simulink model "Tracking"  (R2024b)
settings: Solver=VariableStepAuto  StartTime=0.0  StopTime=1000  RelTol=1e-3
values from neighbouring files (symbols this model uses):
  A = A + DCM_out_slew(:,:,jj)    [sadcode.m]
  a = 6899750    [sadcode.m]
  Area_vect = [3;3;3;3;1;1;1;1;1;1]    [sadcode.m]
  C_d = 2.2    [sadcode.m]
  e = 0.0005895    [sadcode.m]
  G = 6.67e-11    [sadcode.m]
  g = [g1_0 g2_0 g3_0 g4_0 g5_0 g6_0 g7_0 g8_0 g9_0 g10_0  g11_0  g12_0  g13_0 ... (first row only)    [IGRF13.m]
  h = [h1_0 h2_0 h3_0 h4_0 h5_0 h6_0 h7_0 h8_0 h9_0 h10_0  h11_0  h12_0  h13_0 ... (first row only)    [IGRF13.m]
  I = diag([Ix,Iy,Iz])    [sadcode.m]
  i = deg2rad(5.0097)    [sadcode.m]
  Ix = 4.208e11*10^(-3-6)    (= 420.8)    [sadcode.m]
  Iy = 4.922e12*10^(-3-6)    (= 4922)    [sadcode.m]
  Iz = 4.399e12*10^(-3-6)    (= 4399)    [sadcode.m]
  J_b = [1 ; 18 ; 5]    [sadcode.m]
  K_slew = diag(K_slew)    [sadcode.m]
  M = 5.97219e24    (= 5.97219e+24)    [sadcode.m]
  Mount = [0 0 1 0 1 0]    [sadcode.m]
  mu = G*M    (= 398345073000000)    [sadcode.m]
  n = sqrt(mu/a^3)    [sadcode.m]
  N_b = [0,0,+1; 0,0,-1; 0,0,1; 0,0,-1;1,0,0 ; -1,0,0; 0,1,0; 0,-1,0; 0,0,1; 0,0,-1]    [sadcode.m]
  n_face = length(rho_s)    [sadcode.m]
  p = a * (1 - e^2)    (= 6899747.60227)    [sadcode.m]
  q = abs(q(:,1))    [sadcode.m]
  R_f = [2.5,0,0; 2.5,0,0; -2.5,0,0; -2.5,0,0; 1,0,0; -1,0,0; 0,1,0; 0,-1,0; 0,0,1; 0,0,-1]    [sadcode.m]
  R_sun = 149597870700    [sadcode.m]
  rho = 3.13e-13    [sadcode.m]
  theta0 = theta0_slew(jj)    [sadcode.m]
  w0x = w_out_slew(1,jj)    [sadcode.m]
  w0y = w_out_slew(2,jj)    [sadcode.m]
  w0z = w_out_slew(3,jj)    [sadcode.m]
  w_earth = 2*pi/(24*3600)    (= 7.27220521664e-05)    [sadcode.m]
undefined symbols (not defined in the file or in its folder): DiscIntNeverNeededParam
libraries: simulink x4
(part 2 of 2)

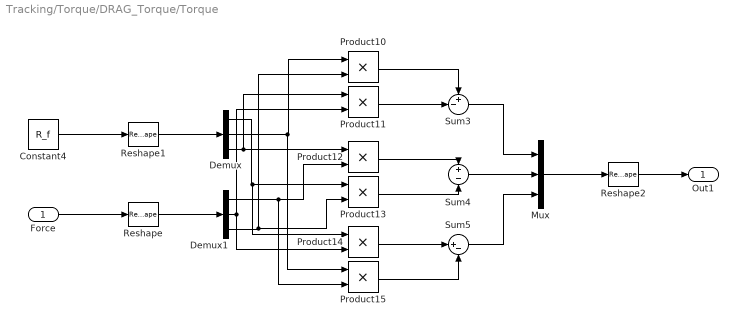
== system Tracking/Torque/DRAG_Torque/Torque ==
  Force : Inport
  Constant4 : Constant  Value=R_f
  Demux : Demux  Outputs=3
  Demux1 : Demux  Outputs=3
  Mux : Mux  Inputs=3
  Product{10..15} (6 alike) : Product
  Reshape : Reshape  OutputDimensionality=Column vector (2-D)
  Reshape1 : Reshape  OutputDimensionality=Column vector (2-D)
  Reshape2 : Reshape  OutputDimensionality=Customize  OutputDimensions=[n_face,3]
  Sum3 : Sum  Inputs=+-|
  Sum4 : Sum  Inputs=+|-
  Sum5 : Sum  Inputs=|+-
  Out1 : Outport
  wires:
  Product12/1 -> Sum4/1
  Demux1/1 -> Product15/2, Product12/2
  Reshape2/1 -> Out1/1
  Demux/1 -> Product14/1, Product13/1
  Sum5/1 -> Mux/3
  Constant4/1 -> Reshape1/1
  Mux/1 -> Reshape2/1
  Reshape/1 -> Demux1/1
  Demux/3 -> Product12/1, Product11/1
  Demux1/3 -> Product13/2, Product10/2
  Force/1 -> Reshape/1
  Product13/1 -> Sum4/2
  Reshape1/1 -> Demux/1
  Sum3/1 -> Mux/1
  Product11/1 -> Sum3/2
  Demux1/2 -> Product11/2, Product14/2
  Demux/2 -> Product15/1, Product10/1
  Sum4/1 -> Mux/2
  Product14/1 -> Sum5/1
  Product10/1 -> Sum3/1
  Product15/1 -> Sum5/2

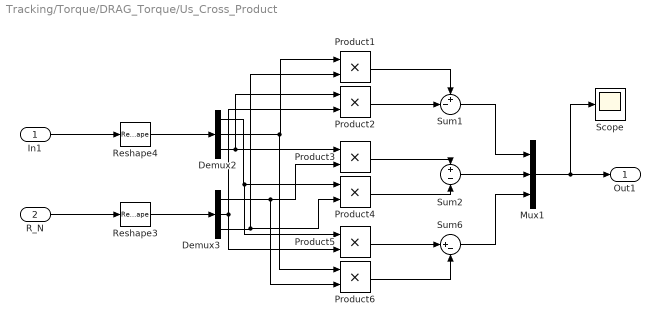
== system Tracking/Torque/DRAG_Torque/Us_Cross_Product  ==
  In1 : Inport
  R_N : Inport  Port=2
  Demux2 : Demux  Outputs=3
  Demux3 : Demux  Outputs=3
  Mux1 : Mux  Inputs=3
  Product{1..6} (6 alike) : Product
  Reshape3 : Reshape  OutputDimensionality=Column vector (2-D)
  Reshape4 : Reshape  OutputDimensionality=Column vector (2-D)
  Scope : Scope
  Sum1 : Sum  Inputs=+-|
  Sum2 : Sum  Inputs=+|-
  Sum6 : Sum  Inputs=|+-
  Out1 : Outport
  wires:
  Reshape3/1 -> Demux3/1
  Reshape4/1 -> Demux2/1
  Demux3/1 -> Product6/2, Product3/2
  Demux2/1 -> Product5/1, Product4/1
  Demux3/3 -> Product4/2, Product1/2
  Sum2/1 -> Mux1/2
  Product6/1 -> Sum6/2
  Sum6/1 -> Mux1/3
  Demux2/2 -> Product6/1, Product1/1
  Demux3/2 -> Product2/2, Product5/2
  Product3/1 -> Sum2/1
  Product2/1 -> Sum1/2
  Product4/1 -> Sum2/2
  Demux2/3 -> Product3/1, Product2/1
  Mux1/1 -> Scope/1, Out1/1
  Product1/1 -> Sum1/1
  Sum1/1 -> Mux1/1
  Product5/1 -> Sum6/1
  In1/1 -> Reshape4/1
  R_N/1 -> Reshape3/1

== system Tracking/Torque/DRAG_Torque/V_vect ==
  Theta : Inport
  Constant : Constant  Value=sqrt(mu/p)
  Constant1 : Constant  Value=e
  Constant2 : Constant  Value=0
  Constant3 : Constant  Value=Rot'
  Gain : Gain  Gain=-1
  Mux : Mux  Inputs=3
  Product : Product
  Product1 : Product  Multiplication=Matrix(*)
  Sin : Trigonometry
  Sin1 : Trigonometry  Operator=cos
  Sum : Sum  Inputs=|++
  Out1 : Outport
  wires:
  Constant/1 -> Product/1
  Mux/1 -> Product/2
  Sin/1 -> Gain/1
  Gain/1 -> Mux/1
  Sin1/1 -> Sum/1
  Sum/1 -> Mux/2
  Constant1/1 -> Sum/2
  Theta/1 -> Sin1/1, Sin/1
  Constant2/1 -> Mux/3
  Constant3/1 -> Product1/1
  Product1/1 -> Out1/1
  Product/1 -> Product1/2

== system Tracking/Torque/GG_Torque/A_BL1 ==
  A_LN : Inport
  A_BN : Inport  Port=2
  Matrix Multiply : Product  Multiplication=Matrix(*)
  Transpose : Math  Operator=transpose
  A_BL : Outport
  wires:
  Transpose/1 -> Matrix Multiply/2
  A_LN/1 -> Transpose/1
  Matrix Multiply/1 -> A_BL/1  "A_BL"
  A_BN/1 -> Matrix Multiply/1

== system Tracking/Torque/GG_Torque/GG_Torque_calc ==
  In1 : Inport
  |R| : Inport  Port=2
  Constant : Constant  Value=G*M
  Constant1 : Constant  Value=3
  Demux : Demux  Outputs=3
  Gain : Gain  Gain=-3
  Multiply3 : Gain  Gain=(Iy-Iz)
  Multiply4 : Gain  Gain=(-Ix+Iz)
  Multiply5 : Gain  Gain=(-Iy+Ix)
  Mux : Mux  Inputs=3
  Product3 : Product  Inputs=***
  Product4 : Product  Inputs=***
  Product5 : Product  Inputs=***
  Product6 : Product  Inputs=*/
  Scope : Scope
  Square : Math  Operator=pow
  GG_Torque : Outport
  wires:
  Multiply3/1 -> Mux/1
  Mux/1 -> GG_Torque/1
  Multiply4/1 -> Mux/2
  In1/1 -> Demux/1
  Product3/1 -> Multiply3/1
  Gain/1 -> Product5/1, Product4/1, Product3/1
  Demux/2 -> Product3/2, Product5/2
  Demux/3 -> Product3/3, Product4/3
  Product4/1 -> Multiply4/1
  Demux/1 -> Product4/2, Product5/3
  Product5/1 -> Multiply5/1
  Product6/1 -> Gain/1
  Constant/1 -> Product6/1
  |R|/1 -> Square/1
  Constant1/1 -> Square/2
  Square/1 -> Scope/1, Product6/2
  Multiply5/1 -> Mux/3

== system Tracking/Torque/GG_Torque/Subsystem ==
  A_BL : Inport
  Constant1 : Constant  Value=[1;0;0]
  Matrix Multiply3 : Product  Multiplication=Matrix(*)
  c_vector : Outport
  wires:
  Constant1/1 -> Matrix Multiply3/2
  Matrix Multiply3/1 -> c_vector/1  "c_vector"
  A_BL/1 -> Matrix Multiply3/1

== system Tracking/Torque/MAG_Torque/Us_Cross_Product ==
  In1 : Inport
  In2 : Inport  Port=2
  Demux2 : Demux  Outputs=3
  Demux3 : Demux  Outputs=3
  Mux1 : Mux  Inputs=3
  Product{1..6} (6 alike) : Product
  Reshape3 : Reshape  OutputDimensionality=Column vector (2-D)
  Reshape4 : Reshape  OutputDimensionality=Column vector (2-D)
  Sum1 : Sum  Inputs=+-|
  Sum2 : Sum  Inputs=+|-
  Sum6 : Sum  Inputs=|+-
  Out1 : Outport
  wires:
  Reshape3/1 -> Demux3/1
  Reshape4/1 -> Demux2/1
  Demux3/1 -> Product6/2, Product3/2
  Demux2/1 -> Product5/1, Product4/1
  Demux3/3 -> Product4/2, Product1/2
  Sum2/1 -> Mux1/2
  Product6/1 -> Sum6/2
  Sum6/1 -> Mux1/3
  Demux2/2 -> Product6/1, Product1/1
  Demux3/2 -> Product2/2, Product5/2
  Product3/1 -> Sum2/1
  Product2/1 -> Sum1/2
  Product4/1 -> Sum2/2
  Demux2/3 -> Product3/1, Product2/1
  Mux1/1 -> Out1/1
  Product1/1 -> Sum1/1
  Sum1/1 -> Mux1/1
  Product5/1 -> Sum6/1
  In1/1 -> Reshape4/1
  In2/1 -> Reshape3/1

== system Tracking/Torque/DRAG_Torque/Force/normalize2 ==
  vector : Inport
  Demux : Demux  Outputs=3
  Product : Product  Inputs=*/
  Square : Math  Operator=square
  Square Root : Sqrt
  Square1 : Math  Operator=square
  Square2 : Math  Operator=square
  Sum : Sum  Inputs=+++
  vers : Outport
  norm : Outport  Port=2
  wires:
  Square Root/1 -> norm/1, Product/2
  Demux/3 -> Square2/1
  Square2/1 -> Sum/3
  Square/1 -> Sum/1
  Square1/1 -> Sum/2
  Demux/1 -> Square/1
  Sum/1 -> Square Root/1
  vector/1 -> Product/1, Demux/1
  Demux/2 -> Square1/1
  Product/1 -> vers/1

== matlab function Tracking/Subsystem5/pseudoinverse ==
  data: u input; y output
function y = fcn(u)
A = u;
% Soluzione con norma minima
x = pinv(A) ;
y = x;

== matlab function Tracking/Torque/MAG_Torque/MATLAB Function1 ==
  data: r_N input; B_N output; t input; g input; h input
function B_N= fcn(r_N,t,g,h)
[B_N]  = earthmagfield13(r_N/1000, t, g, h, 0, 13);%m->km correction
end
